simulink model "Es5_simulink"  (R2025b)
settings: Solver=VariableStepAuto  StartTime=0.0  StopTime=10.0  RelTol=1e-3
undefined symbols (not defined in the file): cos_amp
libraries: simulink x1
settings Model: Creator=fsisa  LastModifiedBy=fsisa

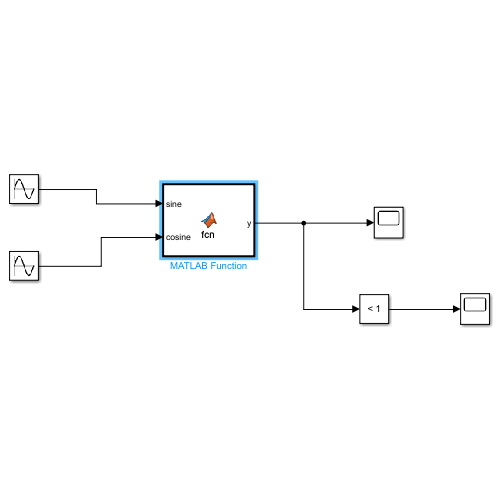
[thumbnail: Simulink's stored preview of the top-level diagram]
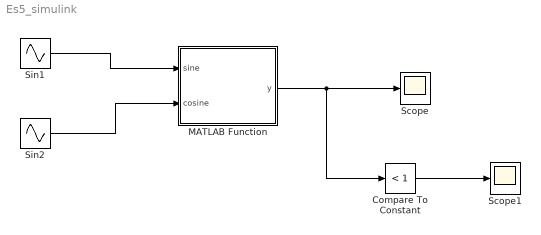
== system Es5_simulink ==
  Compare To Constant : simulink/Logic and Bit Operations/Compare To Constant  relop=<  const=1  OutDataTypeStr=boolean
  MATLAB Function : MATLAB Function  TreatAsAtomicUnit=on
  Scope : Scope
      settings: ActiveDisplayYMinimum=-2.7923888922747118  ActiveDisplayYMaximum=2.7840831284873304
  Scope1 : Scope
      settings: ActiveDisplayYMinimum=-0.12499999999999997  ActiveDisplayYMaximum=1.125
  Sin1 : Sin  SampleTime=0
  Sin2 : Sin  Amplitude=cos_amp  Phase=pi/2  SampleTime=0
  wires:
  Sin2/1 -> MATLAB Function/2(cosine)
  Sin1/1 -> MATLAB Function/1(sine)
  MATLAB Function/1(y) -> Compare To Constant/1, Scope/1
  Compare To Constant/1 -> Scope1/1

== matlab function Es5_simulink/MATLAB Function ==
  data: sine input; y output; cosine input
function y = fcn(sine, cosine)

y = sine - cosine;
